simulink model "sm_car_"  (R2026b)
settings: Solver=ode23t  StopTime=100  MaxStep=0.4  AbsTol=1e-3  EnableMultiTasking=on
PreLoadFcn:
  | % Due to usability issue in Repeating Sequence block
  | warning('off','Simulink:Masking:Invalid');
  | 
  | % Eliminate unnecessary warnings in inactive variants
  | % Warnings generated only if you click through inactive variant
  | warning('off','MATLAB:nonExistentField');
  | warning('off','Simulink:Parameters:BlkParamUndefined');
PostLoadFcn:
  | set_param([bdroot '/Vehicle'],'popup_trailer','Off')
  | warning('off','sm:sli:setup:compile:LocalSolverNotSupported')
  | %sm_car_config_maneuver(bdroot,'WOT Braking');
  | sm_car_config_vehicle(bdroot,'false');
  | sm_car_config_logging(bdroot);
InitFcn:
  | sm_car_config_camera;
  | Vehicle = sm_car_vehcfg_checkConfig(Vehicle);
  | sm_car_check_tire_model(bdroot);
StartFcn:
  | tic;
StopFcn:
  | Elapsed_Sim_Time = toc;
  | % disp(['Elapsed Sim Time = ' num2str(Elapsed_Sim_Time)]);
undefined symbols (not defined in the file or in its folder): acc_theta, accel_ramp_rate, Axle1D, AxleIn, Camera, Control, Driver, Init, Maneuver, Pedal, Scene, ShaftL1, ShaftL2, ShaftR1, ShaftR2, Visual, X, xy_data_car_side, Y, Z
libraries: sm_lib x290, fl_lib x171, nesl_utility x144, simulink x60, simulink_extras x14, sdl_lib x14, SimscapeFluids_lib x7, Damper_Element x4, Tire_1x2x x4, ee_lib x3, Scene_Utilities x3, sharedTrackingLibrary x2
(part 22 of 22)

== matlab function sm_car_/Driver/Closed Loop/Maneuver/MATLAB Function ==
  data: ad output; ref_z output; ref_x output; ref_y output; ref_ayaw output; vTarget output; cp output; p input; q input; posx input; posy input; posz input; xywin input; speed input; yaw input; dist input; pd input; maxld input; minSpd input; speedGain input; ld output; idx_ptMin output; simres output; idx_ptMin_prev input
function [ad,ref_z,ref_x,ref_y,ref_ayaw,vTarget,cp,ld, idx_ptMin, simres] = getPoseCurRef(p,q,posx,posy,posz,xywin,speed,yaw,dist,pd, maxld, minSpd, speedGain, idx_ptMin_prev)

% This function determines the target pose for the vehicle.  It
% interpolates within the provided trajectory to determine the target
% x-y position, yaw angle, and speed. The targets are defined with respect
% to distance along the target trajectory.  The first portion of the
% function determines the distance along the trajectory that the vehicle
% has traveled (ad).  Once that is found, the function interpolates to find
% the target pose at the preview distance (ad+pd).

npts = length(posx);

% Look for nearest point in a window near last evaluation
% Obtain window
if (idx_ptMin_prev == -1)
    % For first evaluation, use entire list of points
    ptlist = 1:npts;
elseif((idx_ptMin_prev-xywin)<1)
    % Window overlaps at lower end: take points from upper end
    win2 = (npts+idx_ptMin_prev-xywin):1:npts;
    win1 = 1:(idx_ptMin_prev+xywin);
    ptlist = [win1 win2];
elseif((idx_ptMin_prev+xywin)>npts)
    % Window overlaps at upper end: take points from lower end
    win2 = (idx_ptMin_prev-xywin):1:npts;
    win1 = 1:(idx_ptMin_prev+xywin-npts);
    ptlist = [win1 win2];
else
    % No overlap: use window
    ptlist = (idx_ptMin_prev-xywin):1:(idx_ptMin_prev+xywin);
end

% Find closest supplied trajectory point to current car position
distances = hypot(p(1) - posx,p(2) - posy);
distances_srch = distances(ptlist);
[~, idx_ptlist] = min(distances_srch);
idx_ptMin = ptlist(idx_ptlist);

%% Identify two trajectory points ahead of and behind closest supplied point
% A, B, C (closest), D, E
idx_ptC = idx_ptMin;
idx_ptA = idx_ptMin-2;
idx_ptB = idx_ptMin-1;
idx_ptD = idx_ptMin+1;
idx_ptE = idx_ptMin+2;

% If we are at end of trajectory, wrap point index
if (idx_ptA<=0),   idx_ptA = idx_ptA+npts; end
if (idx_ptB<=0),   idx_ptB = idx_ptB+npts; end
if (idx_ptD>npts), idx_ptD = idx_ptD-npts; end
if (idx_ptE>npts), idx_ptE = idx_ptE-npts; end

% Extract trajectory point x-y locations
ptA = [posx(idx_ptA); posy(idx_ptA)];
ptB = [posx(idx_ptB); posy(idx_ptB)];
ptC = [posx(idx_ptC); posy(idx_ptC)];
ptD = [posx(idx_ptD); posy(idx_ptD)];
ptE = [posx(idx_ptE); posy(idx_ptE)];

%% Find line separating trajectory segments BC, CD
% Find angle of line connecting BD
qBD = atan2(ptD(2)-ptB(2),ptD(1)-ptB(1));

% Angle of line separating BC, CD is normal to that line
qC  = qBD+pi/2;

%% Determine if we are nearest to trajectory segment BC or BD
% Check if vehicle location and point B on same side of line
% separating segments BC and BD
segBC = arePointsOnSameSide(ptC(1), ptC(2), tan(qC), p(1), p(2), ptB(1), ptB(2));

%% Find vehicle line segment 
% Segment is parallel to closest trajectory segment on which vehicle lies
if(segBC)
   % Use segment BC
   % Line dividing segments AB and BC is normal to line AC 
   qR = atan2(ptC(2)-ptA(2),ptC(1)-ptA(1))+pi/2;
   % Line dividing segments BC and CD has already been found 
   qF = qC;

   ptR = ptB;  % Rear point of segment is point B
   ptF = ptC;  % Front point of segment is point C

   % Angle of vehicle line segment is same as angle of segment BC
   qV = atan2(ptC(2)-ptB(2),ptC(1)-ptB(1));
    % Distance along trajectory to rear of segment
   distR    = dist(idx_ptB);
else
   % Use segment CD
   % Line dividing segments BC and CD has already been found 
   qR = qC;
   % Line dividing segments CD and DE is normal to line CE 
   qF = atan2(ptE(2)-ptC(2),ptE(1)-ptC(1))+pi/2;

   ptR = ptC;    % Rear point of segment is point B
   ptF = ptD;    % Front point of segment is point C

   % Angle of vehicle line segment is same as angle of segment CD
   qV = atan2(ptD(2)-ptC(2),ptD(1)-ptC(1));
    % Distance along trajectory to rear of segment
   distR = dist(idx_ptC);
end

% Length of trajectory segment
distSeg  = sqrt((ptF(1)-ptR(1))^2+(ptF(2)-ptR(2))^2);

% Find endpoints of vehicle line segment
[xR, yR] = findIntersection(p(1), p(2), tan(qV), ptR(1), ptR(2), tan(qR));
[xF, yF] = findIntersection(p(1), p(2), tan(qV), ptF(1), ptF(2), tan(qF));

% Length of vehicle line segment
distFR = sqrt((xR-xF)^2+(yR-yF)^2);
% Distance of vehicle location from rear of vehicle line segment
distvR = sqrt((xR-p(1))^2+(yR-p(2))^2);

% Percentage of distance from vehicle to rear of vehicle line segment 
% Do not permit percentage to go above 100%
% Occurs when vehicle is far from line on inside of curve
segPcnt = min(distvR/distFR,1);

% Distance along trajectory = 
%   Distance to rear of trajectory segment + 
%   length of closest trajectory segment * 
%   percent of vehicle line segment already completed
ad = distR+segPcnt*distSeg;

% Find angle between vehicle location, forward point, and track trajectory
vec_F2v  = ptF - [p(1); p(2)];
vec_F2R  = ptF - ptR;

% Use cosine formula to obtain angle
cos_ang_new = dot(vec_F2v,vec_F2R)/(norm(vec_F2v)*norm(vec_F2R));

% Bound cosine of angle between eps and 1
cos_ang_new = max(cos_ang_new,eps);
cos_ang_new = min(cos_ang_new,1-eps);

% Use angle to obtain lateral distance of vehicle from trajectory
ld = norm(vec_F2v)*sin(acos(cos_ang_new));

% Pose targets for Stanley controller (distance cumulatively sums)
dist4interp = [-dist(end)+dist(1:end-1); dist; dist(end)+dist(2:end)];
posx4interp = [           posx(1:end-1); posx;           posx(2:end)];
posy4interp = [           posy(1:end-1); posy;           posy(2:end)];
posz4interp = [           posz(1:end-1); posz;           posz(2:end)];
speed4interp= [          speed(1:end-1);speed;          speed(2:end)];
% Wrap the interpolation vector for yaw.  
% Necessary to avoid obtaining values between yaw(end) and yaw(1)
yaw4interp  = [-(yaw(end)-yaw(1)) + yaw(1:end-1);  yaw;  (yaw(end)-yaw(1))+ yaw(2:end)];

% Current point
cp = [p(1);p(2);q(3)*180/pi]';

% Reference point obtained from supplied trajectory
% Interpolate using Actual distance (ad) + preview distance (pd)
ref_x    = interp1(dist4interp,posx4interp,ad+pd,'pchip');
ref_y    = interp1(dist4interp,posy4interp,ad+pd,'pchip');
ref_ayaw = interp1(dist4interp,yaw4interp, ad+pd,'pchip');

% For visualization only
ref_z    = interp1(dist4interp,posz4interp,ad+pd);

% Reference velocity obtained from supplied trajectory
% Interpolate using actual distance
vx_cp = interp1(dist4interp,speed4interp,ad);

% Protect for NaNs
ref_x(isnan(ref_x)) = 0;
ref_y(isnan(ref_y)) = 0;
ref_ayaw(isnan(ref_ayaw)) = 0;
ref_z(isnan(ref_z)) = 0;

% Scale speed target
% Reduce speed target if car is far from the target trajectory
if ld < maxld
    vTarget = vx_cp * speedGain;
else
    vTarget = minSpd;
end

% Outputs for debugging calculation
simres = [idx_ptA idx_ptB idx_ptC idx_ptD idx_ptE qC segBC segPcnt xR yR  xF yF p(1) p(2) ad distR distSeg];

end

function [x_intersect, y_intersect] = findIntersection(x1, y1, m1, x2, y2, m2)
    % Check if the slopes are equal (parallel lines)
    if m1 == m2
        error('Invalid trajectory points. The lines are parallel and do not intersect.');
    end
    
    % Calculate the intersection point
    x_intersect = (y2 - y1 + m1*x1 - m2*x2) / (m1 - m2);
    y_intersect = m1 * (x_intersect - x1) + y1;
end

function same_side = arePointsOnSameSide(x0, y0, m, x1, y1, x2, y2)
    % Calculate the line coefficients
    a = -m; % Coefficient of x
    b = 1;  % Coefficient of y
    c = m*x0 - y0; % Constant term
    
    % Calculate the line equation value for both points
    value1 = a*x1 + b*y1 + c;
    value2 = a*x2 + b*y2 + c;
    
    % Check if both values have the same sign
    same_side = (value1 * value2) > 0;
end

== matlab function sm_car_/Driver/Closed Loop1/Maneuver/MATLAB Function ==
  data: ref_z output; ad output; ref_x output; ref_y output; ref_ayaw output; vTarget output; ld output; cp output; simres output; pp_preview_x_pts output; pp_preview_y_pts output; pp_preview_yaw_pts output; pp_preview_dist_pts output; pp_preview_speed_pts output; idx_ptMin output; p input; q input; posx input; posy input; posz input; speed input; xywin input; yaw input; dist input; pd input; maxld input; minSpd input; speedGain input; idx_ptMin_prev input; nPreviewPoints parameter
function [ref_z,ad,ref_x,ref_y,ref_ayaw,vTarget,ld,cp,  simres, ...
          pp_preview_x_pts, pp_preview_y_pts, pp_preview_yaw_pts, pp_preview_dist_pts, pp_preview_speed_pts,idx_ptMin] = ...
          getPoseCurRef(p,q,posx,posy,posz,speed,xywin,yaw,dist,pd, ...
                        maxld, minSpd, speedGain, idx_ptMin_prev, nPreviewPoints)

% This function determines the target pose for the vehicle.  It
% interpolates within the provided trajectory to determine the target
% x-y position, yaw angle, and speed. The targets are defined with respect
% to distance along the target trajectory.  The first portion of the
% function determines the distance along the trajectory that the vehicle
% has traveled (ad).  Once that is found, the function interpolates to find
% the target pose at the preview distance (ad+pd).

npts = length(posx);

% Look for nearest point in a window near last evaluation
% Obtain window
if (idx_ptMin_prev == -1)
    % For first evaluation, use entire list of points
    ptlist = 1:npts;
elseif((idx_ptMin_prev-xywin)<1)
    % Window overlaps at lower end: take points from upper end
    win2 = (npts+idx_ptMin_prev-xywin):1:npts;
    win1 = 1:(idx_ptMin_prev+xywin);
    ptlist = [win1 win2];
elseif((idx_ptMin_prev+xywin)>npts)
    % Window overlaps at upper end: take points from lower end
    win2 = (idx_ptMin_prev-xywin):1:npts;
    win1 = 1:(idx_ptMin_prev+xywin-npts);
    ptlist = [win1 win2];
else
    % No overlap: use window
    ptlist = (idx_ptMin_prev-xywin):1:(idx_ptMin_prev+xywin);
end

% Find closest supplied trajectory point to current car position
distances = hypot(p(1) - posx,p(2) - posy);
distances_srch = distances(ptlist);
[~, idx_ptlist] = min(distances_srch);
idx_ptMin = ptlist(idx_ptlist);

%% Identify two trajectory points ahead of and behind closest supplied point
% A, B, C (closest), D, E
idx_ptC = idx_ptMin;
idx_ptA = idx_ptMin-2;
idx_ptB = idx_ptMin-1;
idx_ptD = idx_ptMin+1;
idx_ptE = idx_ptMin+2;

% If we are at end of trajectory, wrap point index
if (idx_ptA<=0),   idx_ptA = idx_ptA+npts; end
if (idx_ptB<=0),   idx_ptB = idx_ptB+npts; end
if (idx_ptD>npts), idx_ptD = idx_ptD-npts; end
if (idx_ptE>npts), idx_ptE = idx_ptE-npts; end

% Extract trajectory point x-y locations
ptA = [posx(idx_ptA); posy(idx_ptA)];
ptB = [posx(idx_ptB); posy(idx_ptB)];
ptC = [posx(idx_ptC); posy(idx_ptC)];
ptD = [posx(idx_ptD); posy(idx_ptD)];
ptE = [posx(idx_ptE); posy(idx_ptE)];

%% Find line separating trajectory segments BC, CD
% Find angle of line connecting BD
qBD = atan2(ptD(2)-ptB(2),ptD(1)-ptB(1));

% Angle of line separating BC, CD is normal to that line
qC  = qBD+pi/2;

%% Determine if we are nearest to trajectory segment BC or BD
% Check if vehicle location and point B on same side of line
% separating segments BC and BD
segBC = arePointsOnSameSide(ptC(1), ptC(2), tan(qC), p(1), p(2), ptB(1), ptB(2));

%% Find vehicle line segment 
% Segment is parallel to closest trajectory segment on which vehicle lies
if(segBC)
   % Use segment BC
   % Line dividing segments AB and BC is normal to line AC 
   qR = atan2(ptC(2)-ptA(2),ptC(1)-ptA(1))+pi/2;
   % Line dividing segments BC and CD has already been found 
   qF = qC;

   ptR = ptB;  % Rear point of segment is point B
   ptF = ptC;  % Front point of segment is point C

   % Angle of vehicle line segment is same as angle of segment BC
   qV = atan2(ptC(2)-ptB(2),ptC(1)-ptB(1));
    % Distance along trajectory to rear of segment
   distR    = dist(idx_ptB);
else
   % Use segment CD
   % Line dividing segments BC and CD has already been found 
   qR = qC;
   % Line dividing segments CD and DE is normal to line CE 
   qF = atan2(ptE(2)-ptC(2),ptE(1)-ptC(1))+pi/2;

   ptR = ptC;    % Rear point of segment is point B
   ptF = ptD;    % Front point of segment is point C

   % Angle of vehicle line segment is same as angle of segment CD
   qV = atan2(ptD(2)-ptC(2),ptD(1)-ptC(1));
    % Distance along trajectory to rear of segment
   distR = dist(idx_ptC);
end

% Length of trajectory segment
distSeg  = sqrt((ptF(1)-ptR(1))^2+(ptF(2)-ptR(2))^2);

% Find endpoints of vehicle line segment
[xR, yR] = findIntersection(p(1), p(2), tan(qV), ptR(1), ptR(2), tan(qR));
[xF, yF] = findIntersection(p(1), p(2), tan(qV), ptF(1), ptF(2), tan(qF));

% Length of vehicle line segment
distFR = sqrt((xR-xF)^2+(yR-yF)^2);

% Distance of vehicle location from rear of vehicle line segment
% Handle potential division by zero if distFR is very small (e.g. vehicle exactly on ptR or ptF)
if distFR < 1e-6 
    distvR = 0;
else
    distvR = sqrt((xR-p(1))^2+(yR-p(2))^2);
end

% Percentage of distance from vehicle to rear of vehicle line segment 
% Do not permit percentage to go above 100%
% Occurs when vehicle is far from line on inside of curve
segPcnt = min(distvR/distFR,1);

% Distance along trajectory = 
%   Distance to rear of trajectory segment + 
%   length of closest trajectory segment * 
%   percent of vehicle line segment already completed
ad = distR+segPcnt*distSeg;

% Find angle between vehicle location, forward point, and track trajectory
vec_F2v  = ptF - [p(1); p(2)];
vec_F2R  = ptF - ptR;

% Use cosine formula to obtain angle
cos_ang_new = dot(vec_F2v,vec_F2R)/(norm(vec_F2v)*norm(vec_F2R) + eps); % Add eps for stability

% Bound cosine of angle between eps and 1
cos_ang_new = max(cos_ang_new,eps);
cos_ang_new = min(cos_ang_new,1-eps);

% Use angle to obtain lateral distance of vehicle from trajectory
ld = norm(vec_F2v)*sin(acos(cos_ang_new));

%  Prepare interpolation data (handles wrapping) 
% Ensure dist is monotonically increasing for interp1
if any(diff(dist) <= 0) && npts > 1
    % This case should ideally not happen with well-formed 'dist' arrays.
    % If it does, it indicates an issue with the input trajectory 'dist'.
    % For robustness, one might try to fix it or error out.
    % Here, we'll assume 'dist' is mostly fine and proceed,
    % but interp1 might behave unexpectedly.
    % A simple fix for non-codegen mode could be to use unique:
    % [dist_unique, ia, ~] = unique(dist);
    % posx_unique = posx(ia); ... etc.
    % But this is complex for codegen.
    % The provided dist4interp tries to handle wrapping, which is the main concern.
end

% Pose targets for Stanley controller (distance cumulatively sums)
if npts > 1
    dist4interp = [-dist(end)+dist(1:end-1); dist; dist(end)+dist(2:end)];
    posx4interp = [           posx(1:end-1); posx;           posx(2:end)];
    posy4interp = [           posy(1:end-1); posy;           posy(2:end)];
    posz4interp = [           posz(1:end-1); posz;           posz(2:end)];
    speed4interp= [          speed(1:end-1);speed;          speed(2:end)];
    % Wrap the interpolation vector for yaw.
    % Necessary to avoid obtaining values between yaw(end) and yaw(1)
    yaw4interp  = [-(yaw(end)-yaw(1)) + yaw(1:end-1);  yaw;  (yaw(end)-yaw(1))+ yaw(2:end)];
else % Single point trajectory
    dist4interp = dist;
    posx4interp = posx;
    posy4interp = posy;
    posz4interp = posz;
    speed4interp = speed;
    yaw4interp = yaw;
end

%  Current vehicle pose output 
cp = [p(1) p(2) q(3)*180/pi]'; % q(3) is vehicle yaw in rad, convert to deg for cp

% Reference point obtained from supplied trajectory
% Interpolate using Actual distance (ad) + preview distance (pd)
target_dist_single_ref = ad + pd;
ref_x    = interp1(dist4interp,posx4interp,target_dist_single_ref,'pchip');
ref_y    = interp1(dist4interp,posy4interp,target_dist_single_ref,'pchip');
ref_ayaw = interp1(dist4interp,yaw4interp, target_dist_single_ref,'pchip');
ref_z    = interp1(dist4interp,posz4interp,target_dist_single_ref,'pchip'); % For visualization

% Handle NaNs from interp1 if target_dist_single_ref is outside bounds
% (though wrapped dist4interp should prevent this for cyclic paths if pd is reasonable)
if isnan(ref_x); ref_x = posx(idx_ptMin); end % Fallback to closest raw point
if isnan(ref_y); ref_y = posy(idx_ptMin); end
if isnan(ref_ayaw); ref_ayaw = yaw(idx_ptMin); end
if isnan(ref_z); ref_z = posz(idx_ptMin); end

% Reference velocity obtained from supplied trajectory
% Interpolate using actual distance 
vx_cp_trajectory = interp1(dist4interp,speed4interp,ad);
if isnan(vx_cp_trajectory); vx_cp_trajectory = speed(idx_ptMin); end

% Protect for NaNs
ref_x(isnan(ref_x)) = 0;
ref_y(isnan(ref_y)) = 0;
ref_ayaw(isnan(ref_ayaw)) = 0;
ref_z(isnan(ref_z)) = 0;

% Scale speed target
% Reduce speed target if car is far from the target trajectory
if ld < maxld
    % If near target path, use target speed
    vTarget = vx_cp_trajectory * speedGain;
else
    % If too far off track, drop to slow target speed
    vTarget = sign(vx_cp_trajectory) * minSpd;
end

%  Generate Preview Path Segment for Pure Pursuit 
% The segment will span from 'ad' to 'ad + pd'
% 'pd' input now also defines the length of this preview segment
pp_preview_dist_pts = ad + linspace(0, pd, nPreviewPoints);

% Interpolate to get x, y, yaw for these preview points
pp_preview_x_pts     = interp1(dist4interp, posx4interp, pp_preview_dist_pts, 'pchip');
pp_preview_y_pts     = interp1(dist4interp, posy4interp, pp_preview_dist_pts, 'pchip');
pp_preview_yaw_pts   = interp1(dist4interp, yaw4interp, pp_preview_dist_pts, 'pchip');
pp_preview_speed_pts = interp1(dist4interp, speed4interp, pp_preview_dist_pts, 'pchip'); % Added for vx

% Handle potential NaNs from interpolation (e.g., if pd is too large and goes off-path)
% A simple strategy: fill with the last valid point of the original trajectory or the closest point.
% For robustness, we use the values at idx_ptMin if NaNs occur.
for i = 1:nPreviewPoints
    if isnan(pp_preview_x_pts(i)); pp_preview_x_pts(i) = posx(idx_ptMin); end
    if isnan(pp_preview_y_pts(i)); pp_preview_y_pts(i) = posy(idx_ptMin); end
    if isnan(pp_preview_yaw_pts(i)); pp_preview_yaw_pts(i) = yaw(idx_ptMin); end
    if isnan(pp_preview_speed_pts(i)); pp_preview_speed_pts(i) = speed(idx_ptMin); end % Added for vx
    % pp_preview_dist_pts(i) should not be NaN as it's from linspace
end


% Outputs for debugging calculation
simres = [idx_ptA idx_ptB idx_ptC idx_ptD idx_ptE qC segBC segPcnt xR yR  xF yF p(1) p(2) ad distR distSeg];

end

% Helper functions 
% findIntersection and arePointsOnSameSide should be defined as local functions
% or be on the MATLAB path if they are separate .m files. For a single MATLAB Function
% block, they should be local.

function [x_intersect, y_intersect] = findIntersection(x1, y1, m1, x2, y2, m2)
    %#codegen
    % Check if the slopes are equal (parallel lines)
    if abs(m1 - m2) < 1e-9 % Compare with tolerance
        % Handle parallel lines: for codegen, avoid error(), return NaNs or specific values
        x_intersect = NaN;
        y_intersect = NaN;
        % For critical applications, this case needs careful handling based on requirements.
        % One might assert or use a default behavior.
        %coder.varsize('error_msg'); error('Invalid trajectory points. The lines are parallel and do not intersect.');
        return;
    end
    
    % Calculate the intersection point
    x_intersect = (y2 - y1 + m1*x1 - m2*x2) / (m1 - m2);
    y_intersect = m1 * (x_intersect - x1) + y1;
end

function same_side = arePointsOnSameSide(x0, y0, m, x1, y1, x2, y2)
    %#codegen
    % Calculate the line coefficients for line y - y0 = m(x - x0) => mx - y - (mx0 - y0) = 0
    % a*x + b*y + c = 0
    a = m; 
    b = -1;  
    c = -m*x0 + y0; 
    
    % Calculate the line equation value for both points
    value1 = a*x1 + b*y1 + c;
    value2 = a*x2 + b*y2 + c;
    
    % Check if both values have the same sign (or one is zero)
    % Product > 0 means same sign. Product == 0 means one point is on the line.
    same_side = (value1 * value2) >= 0; % Include points on the line as "same side"
end

== matlab function sm_car_/Controller/TrqVec_FLC_V3/Power Control/State Estimation/UKF/MATLAB Function ==
  data: xhat input; Q output
function Q = fcn(xhat)

vx_safe = max(abs(xhat(1)), 1e-3);

if vx_safe < 1.5
    Q_vy = single(2e-7);
else
    Q_vy = single((1e-4* vx_safe)^2);
end

Q = single(diag([1e-5, Q_vy, 1e-6, 5e-5, 1e-4]));

== matlab function sm_car_/Controller/Default/State Estimation/UKF/MATLAB Function ==
  data: xhat input; Q output
function Q = fcn(xhat)

vx_safe = max(abs(xhat(1)), 1e-3);

if vx_safe < 1.5
    Q_vy = single(2e-7);
else
    Q_vy = single((1e-4* vx_safe)^2);
end

Q = single(diag([1e-5, Q_vy, 1e-6, 5e-5, 1e-4]));

== matlab function sm_car_/Controller/TrqVec 4Motor/Power_TqVec/Torque Vectoring/Calculate Torque Split ==
  data: enable input; max_delta_trq input; max_tq input; tq_l_out output; tq_l input; tq_r input; tq_r_out output; tq_tv input; brk input
function [tq_l_out,tq_r_out] = fcn(enable,max_delta_trq,max_tq,tq_l,tq_r,tq_tv,brk)

% enable: flag to turn on torque vectoring
%         True if steering wheel is turned and non-zero vehicle speed
% brk   : flag to turn on torque vectoring
%         True if not braking


% Limit difference in torque between tires lower of 
% (input parameter) and max/min motor torque
t_lim=min(max_tq-abs(tq_l),max_tq-abs(tq_r));
delta_t=min(max_delta_trq,min(t_lim,abs(tq_tv)))*sign(tq_tv)*enable;

if brk>0 
    % Not braking. Use torque vectoring
    tq_l_out=(tq_l-delta_t)*brk;
    tq_r_out=(tq_r+delta_t)*brk;
else
    % No adjustments due to torque vectoring
    tq_l_out=tq_l;
    tq_r_out=tq_r;
end

== stateflow chart sm_car_/Controller/TrqVec 4Motor/Brake Control/ABS/Valve Control L1/Logic ==
  state Inactive
    entry:
    Mod_State = 1;
    Mod_Dur = 10;
  state Initial_Release
    entry:
    Mod_State = 2;
    Mod_Dur = 10;
  state Initial_Apply
    entry:
    Mod_State = 1;
    Mod_Dur = 6;
  state Release
    entry:
    Mod_State = 2;
    Mod_Dur = 6;
  state Apply
    entry:
    Mod_State = 1;
    Mod_Dur = 2;
  state Hold
    entry:
    Mod_State = 0;
    Mod_Dur = 6;
  (default) -> Inactive
  Apply -> Inactive [order 2] : [vSpdEst <0.1]
  Release -> Inactive [order 2] : [vSpdEst <0.1]
  Inactive -> Initial_Release : [Slip>0.5]
  Initial_Release -> Initial_Apply : [Slip<0.1]
  Release -> Initial_Apply [order 1] : [Slip <0.05]
  Initial_Apply -> Hold [order 2] : [Slip>0.1]
  Initial_Apply -> Apply [order 1] : [after(10,msec)]
  Hold -> Release [order 2] : [Slip > 0.25]
  Hold -> Apply [order 1] : [after(40,msec)]
  Apply -> Hold [order 1] : [Slip > 0.1]
  data: Slip input; Mod_State output; Mod_Dur output; vSpdEst input
